simulink model "FT_Sensor_Lab"  (R2025b)
settings: Solver=FixedStepDiscrete  StartTime=0.0  StopTime=4  FixedStep=0.002  RelTol=1e-3
settings Model: Creator=Compu  LastModifiedBy=Compu

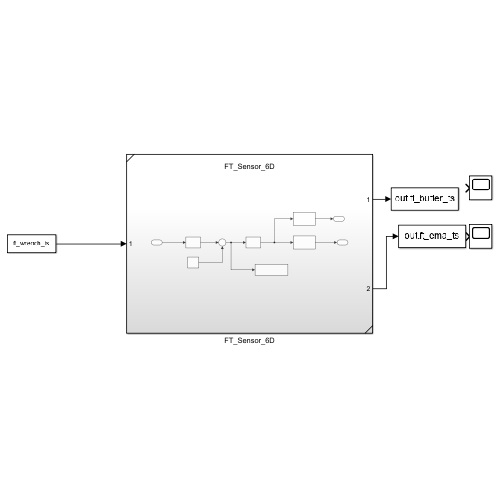
[thumbnail: Simulink's stored preview of the top-level diagram]
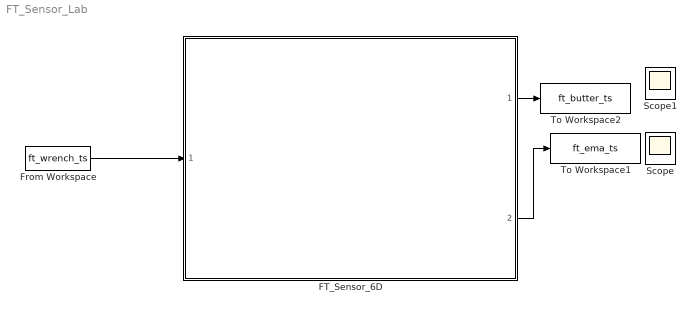
== system FT_Sensor_Lab ==
  FT_Sensor_6D : Subsystem  ReferencedSubsystem=FT_Sensor_6D
  From Workspace : FromWorkspace  VariableName=ft_wrench_ts  SampleTime=0.002  Interpolate=off  OutputAfterFinalValue=Holding final value
  Scope : Scope
      settings: ActiveDisplayYMinimum=-4.0427520972525963  ActiveDisplayYMaximum=6.0514910326547877
  Scope1 : Scope
      settings: ActiveDisplayYMinimum=-1  ActiveDisplayYMaximum=1
  To Workspace1 : ToWorkspace  VariableName=ft_ema_ts  SaveFormat=Timeseries  SampleTime=-1
  To Workspace2 : ToWorkspace  VariableName=ft_butter_ts  SaveFormat=Timeseries  SampleTime=-1
  wires:
  From Workspace/1 -> FT_Sensor_6D/1
  FT_Sensor_6D/1 -> To Workspace2/1
  FT_Sensor_6D/2 -> To Workspace1/1
